simulink model "NILM_Himshikhar_Portal"  (R2026a)
settings: Solver=FixedStepDiscrete  StopTime=10  FixedStep=0.0002
settings Model: Creator=manit  LastModifiedBy=manit

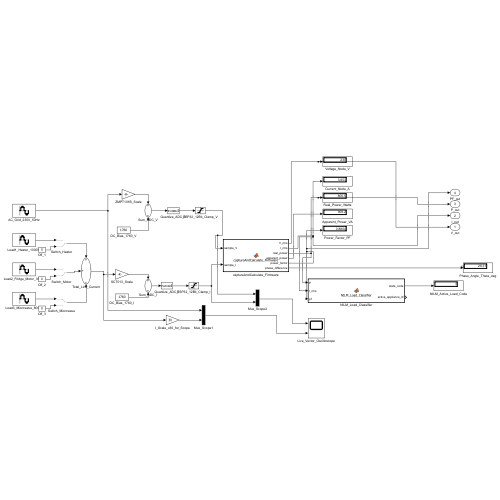
[thumbnail: Simulink's stored preview of the top-level diagram]
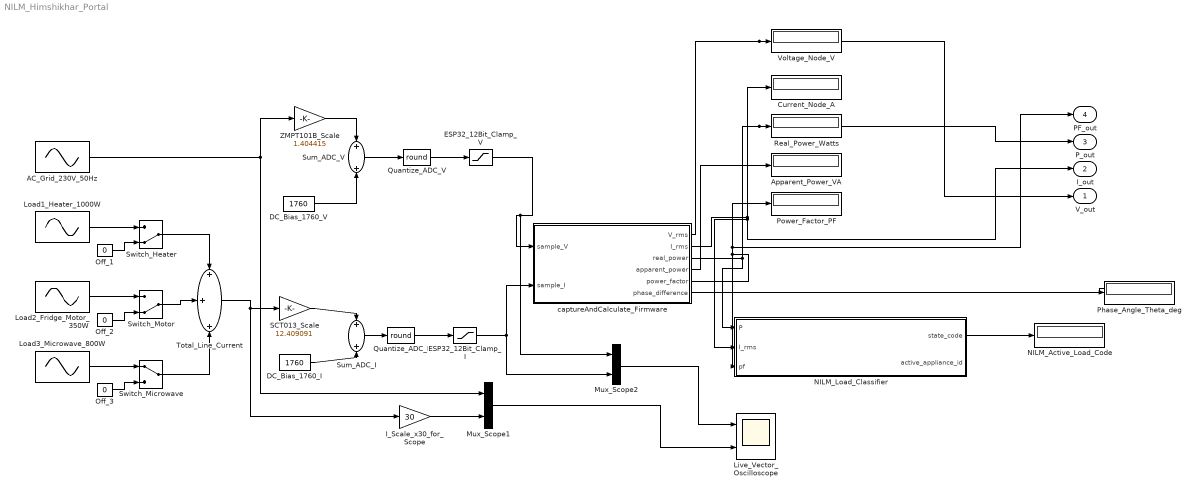
== system NILM_Himshikhar_Portal ==
  AC_Grid_230V_50Hz : Sin  Amplitude=325.2691  Frequency=2*pi*50  SampleTime=0.0002
  Apparent_Power_VA : Display
  Current_Node_A : Display
  DC_Bias_1760_I : Constant  Value=1760
  DC_Bias_1760_V : Constant  Value=1760
  ESP32_12Bit_Clamp_I : Saturate  UpperLimit=4095  LowerLimit=0
  ESP32_12Bit_Clamp_V : Saturate  UpperLimit=4095  LowerLimit=0
  I_Scale_x30_for_Scope : Gain  Gain=30
  Live_Vector_Oscilloscope : Scope  NumInputPorts=2
  Load1_Heater_1000W : Sin  Amplitude=6.1487  Frequency=2*pi*50  SampleTime=0.0002
  Load2_Fridge_Motor_350W : Sin  Amplitude=2.9890  Frequency=2*pi*50  Phase=-0.7679  SampleTime=0.0002
  Load3_Microwave_800W : Sin  Amplitude=5.5898  Frequency=2*pi*50  Phase=-0.4949  SampleTime=0.0002
  Mux_Scope1 : Mux  Inputs=2
  Mux_Scope2 : Mux  Inputs=2
  NILM_Active_Load_Code : Display
  NILM_Load_Classifier : MATLAB Function  TreatAsAtomicUnit=on
  Off_1 : Constant  Value=0
  Off_2 : Constant  Value=0
  Off_3 : Constant  Value=0
  Phase_Angle_Theta_deg : Display
  Power_Factor_PF : Display
  Quantize_ADC_I : Rounding  Operator=round
  Quantize_ADC_V : Rounding  Operator=round
  Real_Power_Watts : Display
  SCT013_Scale : Gain  Gain=12.409091
  Sum_ADC_I : Sum
  Sum_ADC_V : Sum
  Switch_Heater : ManualSwitch  CurrentSetting=0
  Switch_Microwave : ManualSwitch
  Switch_Motor : ManualSwitch  CurrentSetting=0
  Total_Line_Current : Sum  Inputs=+++
  Voltage_Node_V : Display
  ZMPT101B_Scale : Gain  Gain=1.404415
  captureAndCalculate_Firmware : MATLAB Function  TreatAsAtomicUnit=on
  V_out : Outport
  I_out : Outport  Port=2
  P_out : Outport  Port=3
  PF_out : Outport  Port=4
  wires:
  Load1_Heater_1000W/1 -> Switch_Heater/1
  Off_1/1 -> Switch_Heater/2
  Load2_Fridge_Motor_350W/1 -> Switch_Motor/1
  Off_2/1 -> Switch_Motor/2
  Load3_Microwave_800W/1 -> Switch_Microwave/1
  Off_3/1 -> Switch_Microwave/2
  Switch_Heater/1 -> Total_Line_Current/1
  Switch_Motor/1 -> Total_Line_Current/2
  Switch_Microwave/1 -> Total_Line_Current/3
  AC_Grid_230V_50Hz/1 -> Mux_Scope1/1, ZMPT101B_Scale/1
  ZMPT101B_Scale/1 -> Sum_ADC_V/1
  DC_Bias_1760_V/1 -> Sum_ADC_V/2
  Sum_ADC_V/1 -> Quantize_ADC_V/1
  Quantize_ADC_V/1 -> ESP32_12Bit_Clamp_V/1
  Total_Line_Current/1 -> I_Scale_x30_for_Scope/1, SCT013_Scale/1
  SCT013_Scale/1 -> Sum_ADC_I/1
  DC_Bias_1760_I/1 -> Sum_ADC_I/2
  Sum_ADC_I/1 -> Quantize_ADC_I/1
  Quantize_ADC_I/1 -> ESP32_12Bit_Clamp_I/1
  ESP32_12Bit_Clamp_V/1 -> Mux_Scope2/1, captureAndCalculate_Firmware/1(sample_V)
  ESP32_12Bit_Clamp_I/1 -> captureAndCalculate_Firmware/2(sample_I), Mux_Scope2/2
  captureAndCalculate_Firmware/3(real_power) -> P_out/1, Real_Power_Watts/1, NILM_Load_Classifier/1(P)
  captureAndCalculate_Firmware/2(I_rms) -> NILM_Load_Classifier/2(I_rms), Current_Node_A/1, I_out/1
  captureAndCalculate_Firmware/5(power_factor) -> PF_out/1, Power_Factor_PF/1, NILM_Load_Classifier/3(pf)
  captureAndCalculate_Firmware/1(V_rms) -> V_out/1, Voltage_Node_V/1
  captureAndCalculate_Firmware/4(apparent_power) -> Apparent_Power_VA/1
  captureAndCalculate_Firmware/6(phase_difference) -> Phase_Angle_Theta_deg/1
  NILM_Load_Classifier/1(state_code) -> NILM_Active_Load_Code/1
  I_Scale_x30_for_Scope/1 -> Mux_Scope1/2
  Mux_Scope1/1 -> Live_Vector_Oscilloscope/2
  Mux_Scope2/1 -> Live_Vector_Oscilloscope/1

== matlab function NILM_Himshikhar_Portal/NILM_Load_Classifier ==
  data: P input; state_code output; I_rms input; pf input; active_appliance_id output
function [state_code, active_appliance_id] = NILM_Load_Classifier(P, I_rms, pf)
% NILM Non-Intrusive Appliance Classifier
% State 0: No Load / Idle
% State 1: Appliance 1 (Heater, 1000W, PF=1.0)
% State 2: Appliance 2 (Refrigerator Motor, 350W, PF=0.72)
% State 3: Appliance 3 (Microwave, 800W, PF=0.88)
% State 4: Combined Multiple Loads

if (I_rms < 0.5 || P < 50.0)
    state_code = 0; % Idle
    active_appliance_id = 0;
elseif (P >= 900 && P <= 1100 && pf >= 0.96)
    state_code = 1; % Heater alone
    active_appliance_id = 1;
elseif (P >= 280 && P <= 420 && pf >= 0.65 && pf <= 0.78)
    state_code = 2; % Fridge motor alone
    active_appliance_id = 2;
elseif (P >= 720 && P <= 880 && pf >= 0.82 && pf <= 0.92)
    state_code = 3; % Microwave alone
    active_appliance_id = 3;
else
    state_code = 4; % Multiple appliances active
    active_appliance_id = 4;
end

== matlab function NILM_Himshikhar_Portal/captureAndCalculate_Firmware ==
  data: sample_V input; V_rms output; sample_I input; I_rms output; real_power output; apparent_power output; power_factor output; phase_difference output
function [V_rms, I_rms, real_power, apparent_power, power_factor, phase_difference] = captureAndCalculate_Firmware(sample_V, sample_I)
% ESP32 captureAndCalculate() Firmware Implementation
% Constants from user firmware:
VOLTAGE_CAL = 883.58;
CURRENT_CAL = 100.0;
voltage_offset = 1760.0;
current_offset = 1760.0;

% Instantaneous signals:
inst_V = double(sample_V) - voltage_offset;
inst_I = double(sample_I) - current_offset;

% 100ms Temporal Lock Window (N = 500 samples at Ts = 0.0002s):
N = 500;
persistent buf_V_sq buf_I_sq buf_P_inst ptr count_samples
if isempty(ptr)
    buf_V_sq = zeros(1, N);
    buf_I_sq = zeros(1, N);
    buf_P_inst = zeros(1, N);
    ptr = 1;
    count_samples = 0;
end

% Store instantaneous products into window:
buf_V_sq(ptr) = inst_V * inst_V;
buf_I_sq(ptr) = inst_I * inst_I;
buf_P_inst(ptr) = inst_V * inst_I;

ptr = ptr + 1;
if ptr > N
    ptr = 1;
end
if count_samples < N
    count_samples = count_samples + 1;
end

% RMS and Power calculations:
sum_V_squared = sum(buf_V_sq(1:count_samples));
sum_I_squared = sum(buf_I_sq(1:count_samples));
sum_inst_power = sum(buf_P_inst(1:count_samples));
sample_count = count_samples;

V_rms = sqrt(sum_V_squared / sample_count) * (3.3 / 4095.0) * VOLTAGE_CAL;
I_rms = sqrt(sum_I_squared / sample_count) * (3.3 / 4095.0) * CURRENT_CAL;

% Hardware Noise Gates:
if (I_rms < 0.8)
    I_rms = 0.0;
end
if (V_rms < 10.0)
    V_rms = 0.0;
end

real_power = (sum_inst_power / sample_count) * (3.3 / 4095.0)^2 * VOLTAGE_CAL * CURRENT_CAL;
apparent_power = V_rms * I_rms;

if (apparent_power > 5.0)
    power_factor = real_power / apparent_power;
    if (power_factor > 1.0), power_factor = 1.0; end
    if (power_factor < -1.0), power_factor = -1.0; end
    phase_difference = acos(power_factor) * (180.0 / pi);
else
    power_factor = 1.0;
    phase_difference = 0.0;
end
